simulink model "IEEE_BUS_68_AGC"  (R2025a)
settings: Solver=ode23tb  StartTime=0.0  StopTime=150  FixedStep=Ts  MaxStep=0.0001  RelTol=1e-3
PreLoadFcn:
  | PSSMODEL=1;
  | LPSS=0;
  | WAPSS=0;
  | WAPSS2=0;
  | Ts=50e-5;
InitFcn:
  | PSSMODEL=1;
  | LPSS=0;
  | WAPSS=0;
  | WAPSS2=0;
  | Ts=50e-5;
  | 
  | % Required data to 68 Bus benchmark
  | % clear
  | % clc
  | % Definition for the columns
  | % system base =100 MVA
  | 
  | %% Line data Format (line)
  | % All values are given on the same system base MVA
  | % 1: From bus
  | % 2: To bus
  | % 3: Resistance (pu)
  | % 4: Reactance  (pu)
  | % 5: Charge     (pu)
  | % 6: Transformer Tap Amplitute
  | % 7: base MVA
  | % 8: Nomonal Voltage (KV)
  | 
  | %1   2    3        4       5       6        7      8
  | line=[...
  | 1	54	0	     0.0181	  0	      1.025     100    13.8
  | 2	58	0	     0.025	  0	      1.070     100    13.8
  | 3	62	0	     0.02	  0	      1.070     100    13.8
  | 4	19	0.0007	 0.0142	  0	      1.070     100    13.8
  | 5	20	0.0009	 0.018	  0	      1.009     100    13.8
  | 6	22	0	     0.0143	  0	      1.025     100    13.8
  | 7	23	0.0005	 0.0272	  0	      0         100    13.8
  | 8	25	0.0006	 0.0232	  0	      1.025     100    13.8
  | 9	29	0.0008	 0.0156   0	      1.025     100    13.8
  | 10	31	0	     0.026	  0	      1.04      100    13.8
  | 11	32	0	     0.013	  0	      1.04      100    13.8
  | 12	36	0	     0.0075	  0	      1.04      100    13.8
  | 13	17	0	     0.0033	  0	      1.04      100    13.8
  | 14	41	0	     0.0015	  0	      1         100    13.8
  | 15	42	0	     0.0015	  0	      1         100    13.8
  | 16	18	0	     0.003	  0	      1         100    13.8
  | 17	36	0.0005	 0.0045	  0.32	  0         100    138
  | 17	43	0.0005	 0.0276	  0	      0         100    138
  | 18	42	0.004	 0.06	  2.25    0         100    138
  | 18	49	0.0076	 0.1141	  1.16    0	        100    138
  | 18	50	0.0012	 0.0288	  2.06	  0         100    138
  | 20	19	0.0007	 0.0138	  0       1.06	    100    138
  | 19	68	0.0016	 0.0195	  0.304	  0         100    138
  | 21	22	0.0008	 0.014	  0.2565  0	        100    138
  | 21	68	0.0008	 0.0135	  0.2548  0	        100    138
  | 22	23	0.0006	 0.0096	  0.1846  0	        100    138
  | 23	24	0.0022	 0.035	  0.361	  0         100    138
  | 24	68	0.0003	 0.0059	  0.068	  0         100    138
  | 25	26	0.0032	 0.0323	  0.531	  0         100    138
  | 25	54	0.007	 0.0086	  0.146	  0         100    138
  | 26	27	0.0014	 0.0147	  0.2396  0	        100    138
  | 26	28	0.0043	 0.0474	  0.7802  0	        100    138
  | 26	29	0.0057	 0.0625	  1.029	  0         100    138
  | 27	37	0.0013	 0.0173	  0.3216  0	        100    138
  | 27	53	0.032	 0.32	  0.41	  0         100    138
  | ... (+206 lines)
undefined symbols (not defined in the file or in its folder): D1, Delta
libraries: spsPMUPLLBasedPositiveSequenceLib x90, spsRMSLib x73, spsThreePhaseVIMeasurementLib x69, spsLoadFlowBusLib x69, spsThreePhasePISectionLineLib x64, spsThreePhaseParallelRLCLoadLib x35, spsGenericPowerSystemStabilizerLib x32, spsThreePhaseSeriesRLCLoadLib x21, spsThreePhaseTransformerTwoWindingsLib x21, spsSynchronousMachinepuStandardLib x20, spsExcitationSystemLib x16, spsMultiBandPowerSystemStabilizerLib x16
(part 7 of 8)

== system IEEE_BUS_68_AGC/area-5/G15 ==
  "M15: Turbine & Regulators " : Subsystem
  Vref15 : Constant
  gen15 : spsSynchronousMachinepuStandardLib/Synchronous Machine pu Standard  PresetModel=No  MechanicalLoad=Mechanical power Pm  ShowDetailedParameters=on  RotorType=Round  Units=per unit standard parameters  MeasurementBus=off  NominalParameters="[3000*1e6  13.8e3   60 ]"  Reactances1="[mac_con(15,6:8)  mac_con(15,11:13)  mac_con(15,4)]"  Reactances2=[ 1.305, 0.296, 0.252, 0.474, 0.243, 0.18 ]  dAxisTimeConstants=Open-circuit  qAxisTimeConstants=Open-circuit  TimeConstants1=[]  TimeConstants2="[mac_con(15,9:10)  mac_con(15,14:15)]"  TimeConstants3=[]  TimeConstants4=[]  TimeConstants5=[ 1.01, 0.053, 0.1 ]  TimeConstants6=[]  TimeConstants7=[]  TimeConstants8=[]  StatorResistance=mac_con(15,5)  Mechanical="[ mac_con(15,16)  0  4]"  PolePairs=4  InitialConditions=[0 -87.1003 0.333813 0.333813 0.333813 -0.501867 -120.502 119.498 1.00034]  SetSaturation=off  Saturation=[0.6404,0.7127,0.8441,0.9214,0.9956,1.082,1.19,1.316,1.457;0.7,0.7698,0.8872,0.9466,0.9969,1.046,1.1,1.151,1.201]  LoadFlowParameters=[1 830000000 0 0 0]  TsPowergui=0  TsBlock=-1  IterativeModel=Trapezoidal non iterative  IterativeDiscreteModel=Trapezoidal non iterative  BusType=PV  Pref=1000000000  Qref=0  Qmin=-Inf  Qmax=Inf  PLF=0  QLF=0
  A : PMIOPort  Side=Left
  B : PMIOPort  Port=2  Side=Left
  C : PMIOPort  Port=3  Side=Left
  wires:
  "M15: Turbine & Regulators "/1(Pm15) -> gen15/1
  "M15: Turbine & Regulators "/2(Vf15) -> gen15/2
  [PSSmodel] -> "M15: Turbine & Regulators "/4(PSS15)
  Vref15/1 -> "M15: Turbine & Regulators "/3(Vref15)
  gen15/1 -> "M15: Turbine & Regulators "/1(m15)
  [Pref_G15] -> "M15: Turbine & Regulators "/2(Pref15)
  ? -> ?
  ? -> ?
  connections:
  A/RConn1 -- gen15/RConn1
  B/RConn1 -- gen15/RConn2
  C/RConn1 -- gen15/RConn3

== system IEEE_BUS_68_AGC/area-5/G16 ==
  Bus Selector1 : BusSelector  OutputSignals="Mechanical.Rotor speed deviation  dw (pu)"
  "M16: Turbine & Regulators " : Subsystem
  Vref16 : Constant
  gen16 : spsSynchronousMachinepuStandardLib/Synchronous Machine pu Standard  PresetModel=No  MechanicalLoad=Mechanical power Pm  ShowDetailedParameters=on  RotorType=Round  Units=per unit standard parameters  MeasurementBus=off  NominalParameters="[6000*1e6  13.8e3   60 ]"  Reactances1="[mac_con(13,6:8)  mac_con(13,11:13)  mac_con(13,4)]"  Reactances2=[ 1.305, 0.296, 0.252, 0.474, 0.243, 0.18 ]  dAxisTimeConstants=Open-circuit  qAxisTimeConstants=Open-circuit  TimeConstants1=[]  TimeConstants2="[mac_con(13,9:10)  mac_con(13,14:15)]"  TimeConstants3=[]  TimeConstants4=[]  TimeConstants5=[ 1.01, 0.053, 0.1 ]  TimeConstants6=[]  TimeConstants7=[]  TimeConstants8=[]  StatorResistance=mac_con(13,5)  Mechanical="[ mac_con(13,16)  0  4]"  PolePairs=4  InitialConditions=[0 -83.0458 0.584924 0.584924 0.584924 1.77315 -118.227 121.773 1.00142]  SetSaturation=off  Saturation=[0.6404,0.7127,0.8441,0.9214,0.9956,1.082,1.19,1.316,1.457;0.7,0.7698,0.8872,0.9466,0.9969,1.046,1.1,1.151,1.201]  LoadFlowParameters=[1 830000000 0 0 0]  TsPowergui=0  TsBlock=-1  IterativeModel=Trapezoidal non iterative  IterativeDiscreteModel=Trapezoidal non iterative  BusType=PV  Pref=3500000000  Qref=0  Qmin=-Inf  Qmax=Inf  PLF=0  QLF=0
  A : PMIOPort  Side=Left
  B : PMIOPort  Port=2  Side=Left
  C : PMIOPort  Port=3  Side=Left
  tag scope: G16_Goto=global
  wires:
  Vref16/1 -> "M16: Turbine & Regulators "/3(Vref16)
  [PSSmodel] -> "M16: Turbine & Regulators "/4(PSS16)
  "M16: Turbine & Regulators "/2(Vf16) -> gen16/2
  "M16: Turbine & Regulators "/1(Pm16) -> gen16/1
  gen16/1 -> Bus Selector1/1, "M16: Turbine & Regulators "/1(m16)
  Bus Selector1/1 -> [G16_Goto]  "<Rotor speed deviation  dw (pu)>"
  [Pref_G16] -> "M16: Turbine & Regulators "/2(Pref16)
  connections:
  C/RConn1 -- gen16/RConn3
  B/RConn1 -- gen16/RConn2
  A/RConn1 -- gen16/RConn1

== system IEEE_BUS_68_AGC/area-1/gen4/M4: Turbine & Regulators  ==
  note: M4
  m4 : Inport
  Pref4 : Inport  Port=2
  Vref4 : Inport  Port=3
  PSS4 : Inport  Port=4
  Bus Selector : BusSelector  OutputSignals="Mechanical.Rotor speed  wm  (pu),Mechanical.Rotor angle deviation  d_theta (rad),Mechanical.Electrical power  Pe (pu),Mechanical.Rotor speed deviation  dw (pu),Mechanical.Rotor mechanical angle  theta (deg),dq0 components.Stator voltage  vd (pu),dq0 components.Stator voltage  vq (pu),Output reactive power  Qeo (pu)"
  Delta Pa PSS 4 : spsGenericPowerSystemStabilizerLib/Generic Power System Stabilizer  Tsensor=15e-3  K=2.5*1.25  Twashout=1  Tleadlag1=[60e-3 1]  Tleadlag2=[0 0]  VSlimits=[-0.15 0.15]  Vinit=0  Plot_On=off  MagdB_On=on  FreqRange=logspace(-2,2,500)
      settings: LibrarySourceBlock=|
      | sps_lib/Electrical Machines/Synchronous Machine Control/Generic
      | Power System Stabilizer
  Delta w PSS (Kundur) 4 : spsGenericPowerSystemStabilizerLib/Generic Power System Stabilizer  Tsensor=15e-3  K=30  Twashout=10  Tleadlag1=[50e-3 20e-3]  Tleadlag2=[3 5.4]  VSlimits=[-0.15 0.15]  Vinit=0  Plot_On=off  MagdB_On=on  FreqRange=logspace(-2,2,500)
      settings: LibrarySourceBlock=|
      | sps_lib/Electrical Machines/Synchronous Machine Control/Generic
      | Power System Stabilizer
  EXCITATION4 : spsExcitationSystemLib/Excitation System  tr=AVR_Data(4,1)  reg=[ AVR_Data(4,2:3) ]  exc=[ 1, 0 ]  tgr=[ AVR_Data(4,4:5)]  damp=[ 0, 0 ]  sat=[ 0, 0 ]  lim="[ AVR_Data(4,7:8)  0 ]"  v0=[0.997 1.0061]
      settings: LibrarySourceBlock=sps_lib/Electrical Machines/Synchronous Machine Control/Excitation System
  MB-PSS4 : spsMultiBandPowerSystemStabilizerLib/Multi-Band Power System Stabilizer  OperationMode=Simplified settings  Kg=MB(1)  GL=[MB(2) MB(3)]  GI=[MB(4) MB(5)]  GH=[MB(6) MB(7)]  GLd=[66 66 9.4]  TcLF=[1.667 2 0 0 0 0 2 2.4 0 0 0 0 1 1]  GId=[66 66 47.6]  TcIF=[1 1 0.25 0.3 0 0 1 1 0.3 0.36 0 0 0 0]  GHd=[66 66 233]  TcHF="[0.01 0.012 0 0 0 0  0.012 0.0144 0 0 0 0 1 1]"  LIM=[.075 .15 .15 .15]  Plot_On=off  MagdB_On=off  FreqRange=logspace(-2,2,500)
      settings: LibrarySourceBlock=|
      | sps_lib/Electrical Machines/Synchronous Machine Control/Multi-Band
      | Power System Stabilizer
  Multiport Switch1 : MultiPortSwitch  Inputs=4  SaturateOnIntegerOverflow=off
  PSS model3 : Constant  Value=0
  PSS model4 : Constant
  Real-Imag to Complex1 : RealImagToComplex
  STG4 : spsSteamTurbineandGovernorLib/Steam Turbine and Governor  gentype=Tandem-compound (single mass)  reg1="[ 1  0.05    0 ]"  reg2="[ 0.001  0.15 ]"  reg3="[ -0.1  0.1  0  4.496 ]"  N=Ns  turb1="[ 0  10   3.3   0.5   ]"  turb2="[   0   0.36    0.36   0.28   ]"  HA="[ 0.046  1.430  1.465   0.192 ]"  KA="[ 90.44  53.88  64.59   62.94  ]"  DA="[ 0.0115  0.3575  0.3663   0.0137  ]"  ini1=0.632  ini2=[0.779316,-31.4247]
      settings: LibrarySourceBlock=|
      | sps_lib/Electrical Machines/Synchronous Machine Control/Steam Turbine
      | and Governor
  Sum2 : Sum  InputSameDT=on  SaturateOnIntegerOverflow=on  OutDataTypeStr=Inherit: Same as first input
  Sum3 : Sum  Inputs=-+  InputSameDT=on  SaturateOnIntegerOverflow=on  OutDataTypeStr=Inherit: Same as first input
  Terminator3 : Terminator
  Terminator4 : Terminator
  Terminator5 : Terminator
  wref4 : Constant
  Pm4 : Outport  InitialOutput=0
  Vf4 : Outport  Port=2  InitialOutput=0
  tag scope: EFD4=global, Pa4=global, Pe4=global, Q4=global, Vt4=global, d_theta4=global, pss4=global, theta4=global, w4=global
  wires:
  Bus Selector/7 -> EXCITATION4/3, Real-Imag to Complex1/2  "<Stator voltage  vq (pu)>"
  wref4/1 -> STG4/1
  Pref4/1 -> STG4/2
  m4/1 -> Bus Selector/1
  Vref4/1 -> EXCITATION4/1
  EXCITATION4/1 -> Vf4/1, [EFD4]
  Real-Imag to Complex1/1 -> [Vt4]
  Bus Selector/5 -> [theta4]  "<Rotor mechanical angle  theta (deg)>"
  Bus Selector/6 -> EXCITATION4/2, Real-Imag to Complex1/1  "<Stator voltage  vd (pu)>"
  STG4/3 -> Terminator3/1
  STG4/4 -> Sum3/2, Pm4/1
  STG4/2 -> Terminator4/1
  STG4/1 -> Terminator5/1
  Bus Selector/1 -> [w4], STG4/3  "<Rotor speed  wm  (pu)>"
  Bus Selector/2 -> STG4/4, [d_theta4]  "<Rotor angle deviation  d_theta (rad)>"
  Bus Selector/3 -> Sum3/1, [Pe4]  "<Electrical power  Pe (pu)>"
  Bus Selector/4 -> Delta w PSS (Kundur) 4/1, MB-PSS4/1  "<Rotor speed deviation  dw (pu)>"
  Bus Selector/8 -> [Q4]  "<Output reactive power  Qeo (pu)>"
  Sum3/1 -> [Pa4], Delta Pa PSS 4/1  "Pm-Pe"
  Sum2/1 -> Multiport Switch1/1
  PSS model4/1 -> Sum2/2
  Delta Pa PSS 4/1 -> Multiport Switch1/5
  Delta w PSS (Kundur) 4/1 -> Multiport Switch1/4
  MB-PSS4/1 -> Multiport Switch1/3
  PSS model3/1 -> Multiport Switch1/2
  Multiport Switch1/1 -> [pss4], EXCITATION4/4
  PSS4/1 -> Sum2/1

== system IEEE_BUS_68_AGC/area-1/gen5/M5: Turbine & Regulators  ==
  note: M5
  m5 : Inport
  Pref5 : Inport  Port=2
  Vref5 : Inport  Port=3
  PSS5 : Inport  Port=4
  Bus Selector : BusSelector  OutputSignals="Mechanical.Rotor speed  wm  (pu),Mechanical.Rotor angle deviation  d_theta (rad),Mechanical.Electrical power  Pe (pu),Mechanical.Rotor speed deviation  dw (pu),Mechanical.Rotor mechanical angle  theta (deg),dq0 components.Stator voltage  vd (pu),dq0 components.Stator voltage  vq (pu),Output reactive power  Qeo (pu)"
  Delta Pa PSS 5 : spsGenericPowerSystemStabilizerLib/Generic Power System Stabilizer  Tsensor=15e-3  K=2.5*1.25  Twashout=1  Tleadlag1=[60e-3 1]  Tleadlag2=[0 0]  VSlimits=[-0.15 0.15]  Vinit=0  Plot_On=off  MagdB_On=on  FreqRange=logspace(-2,2,500)
      settings: LibrarySourceBlock=|
      | sps_lib/Electrical Machines/Synchronous Machine Control/Generic
      | Power System Stabilizer
  Delta w PSS (Kundur) 5 : spsGenericPowerSystemStabilizerLib/Generic Power System Stabilizer  Tsensor=15e-3  K=30  Twashout=10  Tleadlag1=[50e-3 20e-3]  Tleadlag2=[3 5.4]  VSlimits=[-0.15 0.15]  Vinit=0  Plot_On=off  MagdB_On=on  FreqRange=logspace(-2,2,500)
      settings: LibrarySourceBlock=|
      | sps_lib/Electrical Machines/Synchronous Machine Control/Generic
      | Power System Stabilizer
  EXCITATION5 : spsExcitationSystemLib/Excitation System  tr=AVR_Data(4,1)  reg=[ AVR_Data(4,2:3) ]  exc=[ 1, 0 ]  tgr=[ AVR_Data(4,4:5)]  damp=[ 0, 0 ]  sat=[ 0, 0 ]  lim="[ AVR_Data(4,7:8)  0 ]"  v0=[1.011 1.0593]
      settings: LibrarySourceBlock=sps_lib/Electrical Machines/Synchronous Machine Control/Excitation System
  MB-PSS5 : spsMultiBandPowerSystemStabilizerLib/Multi-Band Power System Stabilizer  OperationMode=Simplified settings  Kg=MB(1)  GL=[MB(2) MB(3)]  GI=[MB(4) MB(5)]  GH=[MB(6) MB(7)]  GLd=[66 66 9.4]  TcLF=[1.667 2 0 0 0 0 2 2.4 0 0 0 0 1 1]  GId=[66 66 47.6]  TcIF=[1 1 0.25 0.3 0 0 1 1 0.3 0.36 0 0 0 0]  GHd=[66 66 233]  TcHF="[0.01 0.012 0 0 0 0  0.012 0.0144 0 0 0 0 1 1]"  LIM=[.075 .15 .15 .15]  Plot_On=off  MagdB_On=off  FreqRange=logspace(-2,2,500)
      settings: LibrarySourceBlock=|
      | sps_lib/Electrical Machines/Synchronous Machine Control/Multi-Band
      | Power System Stabilizer
  Multiport Switch1 : MultiPortSwitch  Inputs=4  SaturateOnIntegerOverflow=off
  PSS model3 : Constant  Value=0
  PSS model4 : Constant
  Real-Imag to Complex1 : RealImagToComplex
  STG5 : spsSteamTurbineandGovernorLib/Steam Turbine and Governor  gentype=Tandem-compound (single mass)  reg1="[ 1  0.05    0 ]"  reg2="[ 0.001  0.15 ]"  reg3="[ -0.1  0.1  0  4.496 ]"  N=Ns  turb1="[ 0  10   3.3   0.5   ]"  turb2="[   0   0.36    0.36   0.28   ]"  HA="[ 0.046  1.430  1.465   0.192 ]"  KA="[ 90.44  53.88  64.59   62.94  ]"  DA="[ 0.0115  0.3575  0.3663   0.0137  ]"  ini1=0.505  ini2=[0.779316,-31.4247]
      settings: LibrarySourceBlock=|
      | sps_lib/Electrical Machines/Synchronous Machine Control/Steam Turbine
      | and Governor
  Sum2 : Sum  InputSameDT=on  SaturateOnIntegerOverflow=on  OutDataTypeStr=Inherit: Same as first input
  Sum3 : Sum  Inputs=-+  InputSameDT=on  SaturateOnIntegerOverflow=on  OutDataTypeStr=Inherit: Same as first input
  Terminator3 : Terminator
  Terminator4 : Terminator
  Terminator5 : Terminator
  wref5 : Constant
  Pm4 : Outport  InitialOutput=0
  Vf5 : Outport  Port=2  InitialOutput=0
  tag scope: EFD5=global, Pa5=global, Pe5=global, Q5=global, Vt5=global, d_theta5=global, pss5=global, theta5=global, w5=global
  wires:
  PSS5/1 -> Sum2/1
  Multiport Switch1/1 -> EXCITATION5/4, [pss5]
  PSS model3/1 -> Multiport Switch1/2
  MB-PSS5/1 -> Multiport Switch1/3
  Delta w PSS (Kundur) 5/1 -> Multiport Switch1/4
  Delta Pa PSS 5/1 -> Multiport Switch1/5
  PSS model4/1 -> Sum2/2
  Sum2/1 -> Multiport Switch1/1
  Sum3/1 -> Delta Pa PSS 5/1, [Pa5]  "Pm-Pe"
  Bus Selector/8 -> [Q5]  "<Output reactive power  Qeo (pu)>"
  Bus Selector/4 -> MB-PSS5/1, Delta w PSS (Kundur) 5/1  "<Rotor speed deviation  dw (pu)>"
  Bus Selector/3 -> [Pe5], Sum3/1  "<Electrical power  Pe (pu)>"
  Bus Selector/2 -> [d_theta5], STG5/4  "<Rotor angle deviation  d_theta (rad)>"
  Bus Selector/1 -> STG5/3, [w5]  "<Rotor speed  wm  (pu)>"
  STG5/1 -> Terminator5/1
  STG5/2 -> Terminator4/1
  STG5/4 -> Pm4/1, Sum3/2
  STG5/3 -> Terminator3/1
  Bus Selector/6 -> Real-Imag to Complex1/1, EXCITATION5/2  "<Stator voltage  vd (pu)>"
  Bus Selector/5 -> [theta5]  "<Rotor mechanical angle  theta (deg)>"
  Real-Imag to Complex1/1 -> [Vt5]
  EXCITATION5/1 -> [EFD5], Vf5/1
  Vref5/1 -> EXCITATION5/1
  m5/1 -> Bus Selector/1
  Pref5/1 -> STG5/2
  wref5/1 -> STG5/1
  Bus Selector/7 -> Real-Imag to Complex1/2, EXCITATION5/3  "<Stator voltage  vq (pu)>"

== system IEEE_BUS_68_AGC/area-1/gen6/M6: Turbine & Regulators  ==
  note: M6
  m6 : Inport
  Pref6 : Inport  Port=2
  Vref6 : Inport  Port=3
  PSS6 : Inport  Port=4
  Bus Selector : BusSelector  OutputSignals="Mechanical.Rotor speed  wm  (pu),Mechanical.Rotor angle deviation  d_theta (rad),Mechanical.Electrical power  Pe (pu),Mechanical.Rotor speed deviation  dw (pu),Mechanical.Rotor mechanical angle  theta (deg),dq0 components.Stator voltage  vd (pu),dq0 components.Stator voltage  vq (pu),Output reactive power  Qeo (pu)"
  Delta Pa PSS 6 : spsGenericPowerSystemStabilizerLib/Generic Power System Stabilizer  Tsensor=15e-3  K=2.5*1.25  Twashout=1  Tleadlag1=[60e-3 1]  Tleadlag2=[0 0]  VSlimits=[-0.15 0.15]  Vinit=0  Plot_On=off  MagdB_On=on  FreqRange=logspace(-2,2,500)
      settings: LibrarySourceBlock=|
      | sps_lib/Electrical Machines/Synchronous Machine Control/Generic
      | Power System Stabilizer
  Delta w PSS (Kundur) 6 : spsGenericPowerSystemStabilizerLib/Generic Power System Stabilizer  Tsensor=15e-3  K=30  Twashout=10  Tleadlag1=[50e-3 20e-3]  Tleadlag2=[3 5.4]  VSlimits=[-0.15 0.15]  Vinit=0  Plot_On=off  MagdB_On=on  FreqRange=logspace(-2,2,500)
      settings: LibrarySourceBlock=|
      | sps_lib/Electrical Machines/Synchronous Machine Control/Generic
      | Power System Stabilizer
  EXCITATION6 : spsExcitationSystemLib/Excitation System  tr=AVR_Data(4,1)  reg=[ AVR_Data(4,2:3) ]  exc=[ 1, 0 ]  tgr=[ AVR_Data(4,4:5)]  damp=[ 0, 0 ]  sat=[ 0, 0 ]  lim="[ AVR_Data(4,7:8)  0 ]"  v0=[1.05 1.103]
      settings: LibrarySourceBlock=sps_lib/Electrical Machines/Synchronous Machine Control/Excitation System
  MB-PSS6 : spsMultiBandPowerSystemStabilizerLib/Multi-Band Power System Stabilizer  OperationMode=Simplified settings  Kg=MB(1)  GL=[MB(2) MB(3)]  GI=[MB(4) MB(5)]  GH=[MB(6) MB(7)]  GLd=[66 66 9.4]  TcLF=[1.667 2 0 0 0 0 2 2.4 0 0 0 0 1 1]  GId=[66 66 47.6]  TcIF=[1 1 0.25 0.3 0 0 1 1 0.3 0.36 0 0 0 0]  GHd=[66 66 233]  TcHF="[0.01 0.012 0 0 0 0  0.012 0.0144 0 0 0 0 1 1]"  LIM=[.075 .15 .15 .15]  Plot_On=off  MagdB_On=off  FreqRange=logspace(-2,2,500)
      settings: LibrarySourceBlock=|
      | sps_lib/Electrical Machines/Synchronous Machine Control/Multi-Band
      | Power System Stabilizer
  Multiport Switch1 : MultiPortSwitch  Inputs=4  SaturateOnIntegerOverflow=off
  PSS model3 : Constant  Value=0
  PSS model4 : Constant
  Real-Imag to Complex1 : RealImagToComplex
  STG6 : spsSteamTurbineandGovernorLib/Steam Turbine and Governor  gentype=Tandem-compound (single mass)  reg1="[ 1  0.05    0 ]"  reg2="[ 0.001  0.15 ]"  reg3="[ -0.1  0.1  0  4.496 ]"  N=Ns  turb1="[ 0  10   3.3   0.5   ]"  turb2="[   0   0.36    0.36   0.28   ]"  HA="[ 0.046  1.430  1.465   0.192 ]"  KA="[ 90.44  53.88  64.59   62.94  ]"  DA="[ 0.0115  0.3575  0.3663   0.0137  ]"  ini1=0.7  ini2=[0.779316,-31.4247]
      settings: LibrarySourceBlock=|
      | sps_lib/Electrical Machines/Synchronous Machine Control/Steam Turbine
      | and Governor
  Sum2 : Sum  InputSameDT=on  SaturateOnIntegerOverflow=on  OutDataTypeStr=Inherit: Same as first input
  Sum3 : Sum  Inputs=-+  InputSameDT=on  SaturateOnIntegerOverflow=on  OutDataTypeStr=Inherit: Same as first input
  Terminator3 : Terminator
  Terminator4 : Terminator
  Terminator5 : Terminator
  wref6 : Constant
  Pm6 : Outport  InitialOutput=0
  Vf6 : Outport  Port=2  InitialOutput=0
  tag scope: EFD6=global, Pa6=global, Pe6=global, Q6=global, Vt6=global, d_theta6=global, pss6=global, theta6=global, w6=global
  wires:
  PSS6/1 -> Sum2/1
  Multiport Switch1/1 -> EXCITATION6/4, [pss6]
  PSS model3/1 -> Multiport Switch1/2
  MB-PSS6/1 -> Multiport Switch1/3
  Delta w PSS (Kundur) 6/1 -> Multiport Switch1/4
  Delta Pa PSS 6/1 -> Multiport Switch1/5
  PSS model4/1 -> Sum2/2
  Sum2/1 -> Multiport Switch1/1
  Sum3/1 -> Delta Pa PSS 6/1, [Pa6]  "Pm-Pe"
  Bus Selector/8 -> [Q6]  "<Output reactive power  Qeo (pu)>"
  Bus Selector/4 -> MB-PSS6/1, Delta w PSS (Kundur) 6/1  "<Rotor speed deviation  dw (pu)>"
  Bus Selector/3 -> [Pe6], Sum3/1  "<Electrical power  Pe (pu)>"
  Bus Selector/2 -> [d_theta6], STG6/4  "<Rotor angle deviation  d_theta (rad)>"
  Bus Selector/1 -> STG6/3, [w6]  "<Rotor speed  wm  (pu)>"
  STG6/1 -> Terminator5/1
  STG6/2 -> Terminator4/1
  STG6/4 -> Pm6/1, Sum3/2
  STG6/3 -> Terminator3/1
  Bus Selector/6 -> Real-Imag to Complex1/1, EXCITATION6/2  "<Stator voltage  vd (pu)>"
  Bus Selector/5 -> [theta6]  "<Rotor mechanical angle  theta (deg)>"
  Real-Imag to Complex1/1 -> [Vt6]
  EXCITATION6/1 -> [EFD6], Vf6/1
  Vref6/1 -> EXCITATION6/1
  m6/1 -> Bus Selector/1
  Pref6/1 -> STG6/2
  wref6/1 -> STG6/1
  Bus Selector/7 -> Real-Imag to Complex1/2, EXCITATION6/3  "<Stator voltage  vq (pu)>"

== system IEEE_BUS_68_AGC/area-1/gen7/M7: Turbine & Regulators  ==
  note: M7
  m7 : Inport
  Pref7 : Inport  Port=2
  Vref7 : Inport  Port=3
  PSS7 : Inport  Port=4
  Bus Selector : BusSelector  OutputSignals="Mechanical.Rotor speed  wm  (pu),Mechanical.Rotor angle deviation  d_theta (rad),Mechanical.Electrical power  Pe (pu),Mechanical.Rotor speed deviation  dw (pu),Mechanical.Rotor mechanical angle  theta (deg),dq0 components.Stator voltage  vd (pu),dq0 components.Stator voltage  vq (pu),Output reactive power  Qeo (pu)"
  Delta Pa PSS 7 : spsGenericPowerSystemStabilizerLib/Generic Power System Stabilizer  Tsensor=15e-3  K=2.5*1.25  Twashout=1  Tleadlag1=[60e-3 1]  Tleadlag2=[0 0]  VSlimits=[-0.15 0.15]  Vinit=0  Plot_On=off  MagdB_On=on  FreqRange=logspace(-2,2,500)
      settings: LibrarySourceBlock=|
      | sps_lib/Electrical Machines/Synchronous Machine Control/Generic
      | Power System Stabilizer
  Delta w PSS (Kundur) 7 : spsGenericPowerSystemStabilizerLib/Generic Power System Stabilizer  Tsensor=15e-3  K=30  Twashout=10  Tleadlag1=[50e-3 20e-3]  Tleadlag2=[3 5.4]  VSlimits=[-0.15 0.15]  Vinit=0  Plot_On=off  MagdB_On=on  FreqRange=logspace(-2,2,500)
      settings: LibrarySourceBlock=|
      | sps_lib/Electrical Machines/Synchronous Machine Control/Generic
      | Power System Stabilizer
  EXCITATION7 : spsExcitationSystemLib/Excitation System  tr=AVR_Data(4,1)  reg=[ AVR_Data(4,2:3) ]  exc=[ 1, 0 ]  tgr=[ AVR_Data(4,4:5)]  damp=[ 0, 0 ]  sat=[ 0, 0 ]  lim="[ AVR_Data(4,7:8)  0 ]"  v0=[1.063 1.1185]
      settings: LibrarySourceBlock=sps_lib/Electrical Machines/Synchronous Machine Control/Excitation System
  MB-PSS7 : spsMultiBandPowerSystemStabilizerLib/Multi-Band Power System Stabilizer  OperationMode=Simplified settings  Kg=MB(1)  GL=[MB(2) MB(3)]  GI=[MB(4) MB(5)]  GH=[MB(6) MB(7)]  GLd=[66 66 9.4]  TcLF=[1.667 2 0 0 0 0 2 2.4 0 0 0 0 1 1]  GId=[66 66 47.6]  TcIF=[1 1 0.25 0.3 0 0 1 1 0.3 0.36 0 0 0 0]  GHd=[66 66 233]  TcHF="[0.01 0.012 0 0 0 0  0.012 0.0144 0 0 0 0 1 1]"  LIM=[.075 .15 .15 .15]  Plot_On=off  MagdB_On=off  FreqRange=logspace(-2,2,500)
      settings: LibrarySourceBlock=|
      | sps_lib/Electrical Machines/Synchronous Machine Control/Multi-Band
      | Power System Stabilizer
  Multiport Switch1 : MultiPortSwitch  Inputs=4  SaturateOnIntegerOverflow=off
  PSS model3 : Constant  Value=0
  PSS model4 : Constant
  Real-Imag to Complex1 : RealImagToComplex
  STG7 : spsSteamTurbineandGovernorLib/Steam Turbine and Governor  gentype=Tandem-compound (single mass)  reg1="[ 1  0.05    0 ]"  reg2="[ 0.001  0.15 ]"  reg3="[ -0.1  0.1  0  4.496 ]"  N=Ns  turb1="[ 0  10   3.3   0.5   ]"  turb2="[   0   0.36    0.36   0.28   ]"  HA="[ 0.046  1.430  1.465   0.192 ]"  KA="[ 90.44  53.88  64.59   62.94  ]"  DA="[ 0.0115  0.3575  0.3663   0.0137  ]"  ini1=0.56  ini2=[0.779316,-31.4247]
      settings: LibrarySourceBlock=|
      | sps_lib/Electrical Machines/Synchronous Machine Control/Steam Turbine
      | and Governor
  Sum2 : Sum  InputSameDT=on  SaturateOnIntegerOverflow=on  OutDataTypeStr=Inherit: Same as first input
  Sum3 : Sum  Inputs=-+  InputSameDT=on  SaturateOnIntegerOverflow=on  OutDataTypeStr=Inherit: Same as first input
  Terminator3 : Terminator
  Terminator4 : Terminator
  Terminator5 : Terminator
  wref7 : Constant
  Pm7 : Outport  InitialOutput=0
  Vf7 : Outport  Port=2  InitialOutput=0
  tag scope: EFD7=global, Pa7=global, Pe7=global, Q7=global, Vt7=global, d_theta7=global, pss7=global, theta7=global, w7=global
  wires:
  PSS7/1 -> Sum2/1
  Multiport Switch1/1 -> EXCITATION7/4, [pss7]
  PSS model3/1 -> Multiport Switch1/2
  MB-PSS7/1 -> Multiport Switch1/3
  Delta w PSS (Kundur) 7/1 -> Multiport Switch1/4
  Delta Pa PSS 7/1 -> Multiport Switch1/5
  PSS model4/1 -> Sum2/2
  Sum2/1 -> Multiport Switch1/1
  Sum3/1 -> Delta Pa PSS 7/1, [Pa7]  "Pm-Pe"
  Bus Selector/8 -> [Q7]  "<Output reactive power  Qeo (pu)>"
  Bus Selector/4 -> MB-PSS7/1, Delta w PSS (Kundur) 7/1  "<Rotor speed deviation  dw (pu)>"
  Bus Selector/3 -> [Pe7], Sum3/1  "<Electrical power  Pe (pu)>"
  Bus Selector/2 -> [d_theta7], STG7/4  "<Rotor angle deviation  d_theta (rad)>"
  Bus Selector/1 -> STG7/3, [w7]  "<Rotor speed  wm  (pu)>"
  STG7/1 -> Terminator5/1
  STG7/2 -> Terminator4/1
  STG7/4 -> Pm7/1, Sum3/2
  STG7/3 -> Terminator3/1
  Bus Selector/6 -> Real-Imag to Complex1/1, EXCITATION7/2  "<Stator voltage  vd (pu)>"
  Bus Selector/5 -> [theta7]  "<Rotor mechanical angle  theta (deg)>"
  Real-Imag to Complex1/1 -> [Vt7]
  EXCITATION7/1 -> [EFD7], Vf7/1
  Vref7/1 -> EXCITATION7/1
  m7/1 -> Bus Selector/1
  Pref7/1 -> STG7/2
  wref7/1 -> STG7/1
  Bus Selector/7 -> Real-Imag to Complex1/2, EXCITATION7/3  "<Stator voltage  vq (pu)>"

== system IEEE_BUS_68_AGC/area-2/G2/M2: Turbine & Regulators  ==
  note: M2
  m2 : Inport
  Pref2 : Inport  Port=2
  Vref2 : Inport  Port=3
  PSS2 : Inport  Port=4
  Bus Selector : BusSelector  OutputSignals="Mechanical.Rotor speed  wm  (pu),Mechanical.Rotor angle deviation  d_theta (rad),Mechanical.Electrical power  Pe (pu),Mechanical.Rotor speed deviation  dw (pu),Mechanical.Rotor mechanical angle  theta (deg),dq0 components.Stator voltage  vd (pu),dq0 components.Stator voltage  vq (pu),Output reactive power  Qeo (pu)"
  "Delta Pa PSS 2 " : spsGenericPowerSystemStabilizerLib/Generic Power System Stabilizer  Tsensor=15e-3  K=2.5*1.25  Twashout=1  Tleadlag1=[60e-3 1]  Tleadlag2=[0 0]  VSlimits=[-0.15 0.15]  Vinit=0  Plot_On=off  MagdB_On=on  FreqRange=logspace(-2,2,500)
      settings: LibrarySourceBlock=|
      | sps_lib/Electrical Machines/Synchronous Machine Control/Generic
      | Power System Stabilizer
  Delta w PSS (Kundur) 2 : spsGenericPowerSystemStabilizerLib/Generic Power System Stabilizer  Tsensor=15e-3  K=30  Twashout=10  Tleadlag1=[50e-3 20e-3]  Tleadlag2=[3 5.4]  VSlimits=[-0.15 0.15]  Vinit=0  Plot_On=off  MagdB_On=on  FreqRange=logspace(-2,2,500)
      settings: LibrarySourceBlock=|
      | sps_lib/Electrical Machines/Synchronous Machine Control/Generic
      | Power System Stabilizer
  EXCITATION2 : spsExcitationSystemLib/Excitation System  tr=AVR_Data(2,1)  reg=[ AVR_Data(2,2:3) ]  exc=[ 1, 0 ]  tgr=[ AVR_Data(2,4:5)]  damp=[ 0, 0 ]  sat=[ 0, 0 ]  lim="[ AVR_Data(2,7:8)  0 ]"  v0=[0.98 1.019]
      settings: LibrarySourceBlock=sps_lib/Electrical Machines/Synchronous Machine Control/Excitation System
  MB-PSS2 : spsMultiBandPowerSystemStabilizerLib/Multi-Band Power System Stabilizer  OperationMode=Simplified settings  Kg=MB(1)  GL=[MB(2) MB(3)]  GI=[MB(4) MB(5)]  GH=[MB(6) MB(7)]  GLd=[66 66 9.4]  TcLF=[1.667 2 0 0 0 0 2 2.4 0 0 0 0 1 1]  GId=[66 66 47.6]  TcIF=[1 1 0.25 0.3 0 0 1 1 0.3 0.36 0 0 0 0]  GHd=[66 66 233]  TcHF="[0.01 0.012 0 0 0 0  0.012 0.0144 0 0 0 0 1 1]"  LIM=[.075 .15 .15 .15]  Plot_On=off  MagdB_On=off  FreqRange=logspace(-2,2,500)
      settings: LibrarySourceBlock=|
      | sps_lib/Electrical Machines/Synchronous Machine Control/Multi-Band
      | Power System Stabilizer
  Multiport Switch1 : MultiPortSwitch  Inputs=4  SaturateOnIntegerOverflow=off
  PSS model3 : Constant  Value=0
  PSS model4 : Constant
  Real-Imag to Complex1 : RealImagToComplex
  STG2 : spsSteamTurbineandGovernorLib/Steam Turbine and Governor  gentype=Tandem-compound (single mass)  reg1="[ 1  0.05    0 ]"  reg2="[ 0.001  0.15 ]"  reg3="[ -0.1  0.1  0  4.496 ]"  N=Ns  turb1="[ 0  10   3.3   0.5   ]"  turb2="[   0   0.36    0.36   0.28   ]"  HA="[ 0.046  1.430  1.465   0.192 ]"  KA="[ 90.44  53.88  64.59   62.94  ]"  DA="[ 0.0115  0.3575  0.3663   0.0137  ]"  ini1=0.545  ini2=[0.779316,-31.4247]
      settings: LibrarySourceBlock=|
      | sps_lib/Electrical Machines/Synchronous Machine Control/Steam Turbine
      | and Governor
  Sum2 : Sum  InputSameDT=on  SaturateOnIntegerOverflow=on  OutDataTypeStr=Inherit: Same as first input
  Sum3 : Sum  Inputs=-+  InputSameDT=on  SaturateOnIntegerOverflow=on  OutDataTypeStr=Inherit: Same as first input
  Terminator3 : Terminator
  Terminator4 : Terminator
  Terminator5 : Terminator
  wref2 : Constant
  Pm2 : Outport  InitialOutput=0
  Vf2 : Outport  Port=2  InitialOutput=0
  tag scope: EFD2=global, Pa2=global, Pe2=global, Q2=global, Vt2=global, d_theta2=global, pss2=global, theta2=global, w2=global
  wires:
  Bus Selector/7 -> EXCITATION2/3, Real-Imag to Complex1/2  "<Stator voltage  vq (pu)>"
  wref2/1 -> STG2/1
  Pref2/1 -> STG2/2
  m2/1 -> Bus Selector/1
  Vref2/1 -> EXCITATION2/1
  EXCITATION2/1 -> Vf2/1, [EFD2]
  Real-Imag to Complex1/1 -> [Vt2]
  Bus Selector/5 -> [theta2]  "<Rotor mechanical angle  theta (deg)>"
  Bus Selector/6 -> EXCITATION2/2, Real-Imag to Complex1/1  "<Stator voltage  vd (pu)>"
  STG2/3 -> Terminator3/1
  STG2/4 -> Sum3/2, Pm2/1
  STG2/2 -> Terminator4/1
  STG2/1 -> Terminator5/1
  Bus Selector/1 -> [w2], STG2/3  "<Rotor speed  wm  (pu)>"
  Bus Selector/2 -> STG2/4, [d_theta2]  "<Rotor angle deviation  d_theta (rad)>"
  Bus Selector/3 -> Sum3/1, [Pe2]  "<Electrical power  Pe (pu)>"
  Bus Selector/4 -> Delta w PSS (Kundur) 2/1, MB-PSS2/1  "<Rotor speed deviation  dw (pu)>"
  Bus Selector/8 -> [Q2]  "<Output reactive power  Qeo (pu)>"
  Sum3/1 -> [Pa2], "Delta Pa PSS 2 "/1  "Pm-Pe"
  Sum2/1 -> Multiport Switch1/1
  PSS model4/1 -> Sum2/2
  "Delta Pa PSS 2 "/1 -> Multiport Switch1/5
  Delta w PSS (Kundur) 2/1 -> Multiport Switch1/4
  MB-PSS2/1 -> Multiport Switch1/3
  PSS model3/1 -> Multiport Switch1/2
  Multiport Switch1/1 -> [pss2], EXCITATION2/4
  PSS2/1 -> Sum2/1

== system IEEE_BUS_68_AGC/area-2/G3/M3: Turbine & Regulators  ==
  note: M3
  m3 : Inport
  Pref3 : Inport  Port=2
  Vref3 : Inport  Port=3
  PSS3 : Inport  Port=4
  Bus Selector : BusSelector  OutputSignals="Mechanical.Rotor speed  wm  (pu),Mechanical.Rotor angle deviation  d_theta (rad),Mechanical.Electrical power  Pe (pu),Mechanical.Rotor speed deviation  dw (pu),Mechanical.Rotor mechanical angle  theta (deg),dq0 components.Stator voltage  vd (pu),dq0 components.Stator voltage  vq (pu),Output reactive power  Qeo (pu)"
  "Delta Pa PSS 3 " : spsGenericPowerSystemStabilizerLib/Generic Power System Stabilizer  Tsensor=15e-3  K=2.5*1.25  Twashout=1  Tleadlag1=[60e-3 1]  Tleadlag2=[0 0]  VSlimits=[-0.15 0.15]  Vinit=0  Plot_On=off  MagdB_On=on  FreqRange=logspace(-2,2,500)
      settings: LibrarySourceBlock=|
      | sps_lib/Electrical Machines/Synchronous Machine Control/Generic
      | Power System Stabilizer
  Delta w PSS (Kundur) 3 : spsGenericPowerSystemStabilizerLib/Generic Power System Stabilizer  Tsensor=15e-3  K=30  Twashout=10  Tleadlag1=[50e-3 20e-3]  Tleadlag2=[3 5.4]  VSlimits=[-0.15 0.15]  Vinit=0  Plot_On=off  MagdB_On=on  FreqRange=logspace(-2,2,500)
      settings: LibrarySourceBlock=|
      | sps_lib/Electrical Machines/Synchronous Machine Control/Generic
      | Power System Stabilizer
  EXCITATION3 : spsExcitationSystemLib/Excitation System  tr=AVR_Data(3,1)  reg=[ AVR_Data(3,2:3) ]  exc=[ 1, 0 ]  tgr=[ AVR_Data(3,4:5)]  damp=[ 0, 0 ]  sat=[ 0, 0 ]  lim="[ AVR_Data(3,7:8)  0 ]"  v0=[0.983 0.98897]
      settings: LibrarySourceBlock=sps_lib/Electrical Machines/Synchronous Machine Control/Excitation System
  MB-PSS3 : spsMultiBandPowerSystemStabilizerLib/Multi-Band Power System Stabilizer  OperationMode=Simplified settings  Kg=MB(1)  GL=[MB(2) MB(3)]  GI=[MB(4) MB(5)]  GH=[MB(6) MB(7)]  GLd=[66 66 9.4]  TcLF=[1.667 2 0 0 0 0 2 2.4 0 0 0 0 1 1]  GId=[66 66 47.6]  TcIF=[1 1 0.25 0.3 0 0 1 1 0.3 0.36 0 0 0 0]  GHd=[66 66 233]  TcHF="[0.01 0.012 0 0 0 0  0.012 0.0144 0 0 0 0 1 1]"  LIM=[.075 .15 .15 .15]  Plot_On=off  MagdB_On=off  FreqRange=logspace(-2,2,500)
      settings: LibrarySourceBlock=|
      | sps_lib/Electrical Machines/Synchronous Machine Control/Multi-Band
      | Power System Stabilizer
  Multiport Switch1 : MultiPortSwitch  Inputs=4  SaturateOnIntegerOverflow=off
  PSS model3 : Constant  Value=0
  PSS model4 : Constant
  Real-Imag to Complex1 : RealImagToComplex
  STG3 : spsSteamTurbineandGovernorLib/Steam Turbine and Governor  gentype=Tandem-compound (single mass)  reg1="[ 1  0.05    0 ]"  reg2="[ 0.001  0.15 ]"  reg3="[ -0.1  0.1  0  4.496 ]"  N=Ns  turb1="[ 0  10   3.3   0.5   ]"  turb2="[   0   0.36    0.36   0.28   ]"  HA="[ 0.046  1.430  1.465   0.192 ]"  KA="[ 90.44  53.88  64.59   62.94  ]"  DA="[ 0.0115  0.3575  0.3663   0.0137  ]"  ini1=0.325  ini2=[0.779316,-31.4247]
      settings: LibrarySourceBlock=|
      | sps_lib/Electrical Machines/Synchronous Machine Control/Steam Turbine
      | and Governor
  Sum2 : Sum  InputSameDT=on  SaturateOnIntegerOverflow=on  OutDataTypeStr=Inherit: Same as first input
  Sum3 : Sum  Inputs=-+  InputSameDT=on  SaturateOnIntegerOverflow=on  OutDataTypeStr=Inherit: Same as first input
  Terminator3 : Terminator
  Terminator4 : Terminator
  Terminator5 : Terminator
  wref3 : Constant
  Pm3 : Outport  InitialOutput=0
  Vf3 : Outport  Port=2  InitialOutput=0
  tag scope: EFD3=global, Pa3=global, Pe3=global, Q3=global, Vt3=global, d_theta3=global, pss3=global, theta3=global, w3=global
  wires:
  PSS3/1 -> Sum2/1
  Multiport Switch1/1 -> EXCITATION3/4, [pss3]
  PSS model3/1 -> Multiport Switch1/2
  MB-PSS3/1 -> Multiport Switch1/3
  Delta w PSS (Kundur) 3/1 -> Multiport Switch1/4
  "Delta Pa PSS 3 "/1 -> Multiport Switch1/5
  PSS model4/1 -> Sum2/2
  Sum2/1 -> Multiport Switch1/1
  Sum3/1 -> "Delta Pa PSS 3 "/1, [Pa3]  "Pm-Pe"
  Bus Selector/8 -> [Q3]  "<Output reactive power  Qeo (pu)>"
  Bus Selector/4 -> MB-PSS3/1, Delta w PSS (Kundur) 3/1  "<Rotor speed deviation  dw (pu)>"
  Bus Selector/3 -> [Pe3], Sum3/1  "<Electrical power  Pe (pu)>"
  Bus Selector/2 -> [d_theta3], STG3/4  "<Rotor angle deviation  d_theta (rad)>"
  Bus Selector/1 -> STG3/3, [w3]  "<Rotor speed  wm  (pu)>"
  STG3/1 -> Terminator5/1
  STG3/2 -> Terminator4/1
  STG3/4 -> Pm3/1, Sum3/2
  STG3/3 -> Terminator3/1
  Bus Selector/6 -> Real-Imag to Complex1/1, EXCITATION3/2  "<Stator voltage  vd (pu)>"
  Bus Selector/5 -> [theta3]  "<Rotor mechanical angle  theta (deg)>"
  Real-Imag to Complex1/1 -> [Vt3]
  EXCITATION3/1 -> [EFD3], Vf3/1
  Vref3/1 -> EXCITATION3/1
  m3/1 -> Bus Selector/1
  Pref3/1 -> STG3/2
  wref3/1 -> STG3/1
  Bus Selector/7 -> Real-Imag to Complex1/2, EXCITATION3/3  "<Stator voltage  vq (pu)>"

== system IEEE_BUS_68_AGC/area-3/G1/M1: Turbine & Regulators  ==
  note: M1
  m1 : Inport
  Pref1 : Inport  Port=2
  Vref1 : Inport  Port=3
  PSS1 : Inport  Port=4
  Bus Selector : BusSelector  OutputSignals="Mechanical.Rotor speed  wm  (pu),Mechanical.Rotor angle deviation  d_theta (rad),Mechanical.Electrical power  Pe (pu),Mechanical.Rotor speed deviation  dw (pu),Mechanical.Rotor mechanical angle  theta (deg),dq0 components.Stator voltage  vd (pu),dq0 components.Stator voltage  vq (pu),Output reactive power  Qeo (pu)"
  "Delta Pa PSS 1 " : spsGenericPowerSystemStabilizerLib/Generic Power System Stabilizer  Tsensor=15e-3  K=2.5*1.25  Twashout=1  Tleadlag1=[60e-3 1]  Tleadlag2=[0 0]  VSlimits=[-0.15 0.15]  Vinit=0  Plot_On=off  MagdB_On=on  FreqRange=logspace(-2,2,500)
      settings: LibrarySourceBlock=|
      | sps_lib/Electrical Machines/Synchronous Machine Control/Generic
      | Power System Stabilizer
  Delta w PSS (Kundur) 1 : spsGenericPowerSystemStabilizerLib/Generic Power System Stabilizer  Tsensor=15e-3  K=30  Twashout=10  Tleadlag1=[50e-3 20e-3]  Tleadlag2=[3 5.4]  VSlimits=[-0.15 0.15]  Vinit=0  Plot_On=off  MagdB_On=on  FreqRange=logspace(-2,2,500)
      settings: LibrarySourceBlock=|
      | sps_lib/Electrical Machines/Synchronous Machine Control/Generic
      | Power System Stabilizer
  EXCITATION1 : spsExcitationSystemLib/Excitation System  tr=AVR_Data(1,1)  reg=[ AVR_Data(1,2:3) ]  exc=[ 1, 0 ]  tgr=[ AVR_Data(1,4:5)]  damp=[ 0, 0 ]  sat=[ 0, 0 ]  lim="[ AVR_Data(1,7:8)  0 ]"  v0=[1.045 1.0597]
      settings: LibrarySourceBlock=sps_lib/Electrical Machines/Synchronous Machine Control/Excitation System
  MB-PSS1 : spsMultiBandPowerSystemStabilizerLib/Multi-Band Power System Stabilizer  OperationMode=Simplified settings  Kg=MB(1)  GL=[MB(2) MB(3)]  GI=[MB(4) MB(5)]  GH=[MB(6) MB(7)]  GLd=[66 66 9.4]  TcLF=[1.667 2 0 0 0 0 2 2.4 0 0 0 0 1 1]  GId=[66 66 47.6]  TcIF=[1 1 0.25 0.3 0 0 1 1 0.3 0.36 0 0 0 0]  GHd=[66 66 233]  TcHF="[0.01 0.012 0 0 0 0  0.012 0.0144 0 0 0 0 1 1]"  LIM=[.075 .15 .15 .15]  Plot_On=off  MagdB_On=off  FreqRange=logspace(-2,2,500)
      settings: LibrarySourceBlock=|
      | sps_lib/Electrical Machines/Synchronous Machine Control/Multi-Band
      | Power System Stabilizer
  Multiport Switch1 : MultiPortSwitch  Inputs=4  SaturateOnIntegerOverflow=off
  PSS model3 : Constant  Value=0
  PSS model4 : Constant
  Real-Imag to Complex1 : RealImagToComplex
  STG1 : spsSteamTurbineandGovernorLib/Steam Turbine and Governor  gentype=Tandem-compound (single mass)  reg1="[ 1  0.05    0 ]"  reg2="[ 0.001  0.15 ]"  reg3="[ -0.1  0.1  0  4.496 ]"  N=Ns  turb1="[ 0  10   3.3   0.5   ]"  turb2="[   0   0.36    0.36   0.28   ]"  HA="[ 0.046  1.430  1.465   0.192 ]"  KA="[ 90.44  53.88  64.59   62.94  ]"  DA="[ 0.0115  0.3575  0.3663   0.0137  ]"  ini1=0.25  ini2=[0.779316,-31.4247]
      settings: LibrarySourceBlock=|
      | sps_lib/Electrical Machines/Synchronous Machine Control/Steam Turbine
      | and Governor
  Sum2 : Sum  InputSameDT=on  SaturateOnIntegerOverflow=on  OutDataTypeStr=Inherit: Same as first input
  Sum3 : Sum  Inputs=-+  InputSameDT=on  SaturateOnIntegerOverflow=on  OutDataTypeStr=Inherit: Same as first input
  Terminator3 : Terminator
  Terminator4 : Terminator
  Terminator5 : Terminator
  wref1 : Constant
  Pm1 : Outport  InitialOutput=0
  Vf1 : Outport  Port=2  InitialOutput=0
  tag scope: EFD1=global, Pa1=global, Pe1=global, Q1=global, Vt1=global, d_theta1=global, pss1=global, theta1=global, w1=global
  wires:
  PSS1/1 -> Sum2/1
  Multiport Switch1/1 -> EXCITATION1/4, [pss1]
  PSS model3/1 -> Multiport Switch1/2
  MB-PSS1/1 -> Multiport Switch1/3
  Delta w PSS (Kundur) 1/1 -> Multiport Switch1/4
  "Delta Pa PSS 1 "/1 -> Multiport Switch1/5
  PSS model4/1 -> Sum2/2
  Sum2/1 -> Multiport Switch1/1
  Sum3/1 -> "Delta Pa PSS 1 "/1, [Pa1]  "Pm-Pe"
  Bus Selector/8 -> [Q1]  "<Output reactive power  Qeo (pu)>"
  Bus Selector/4 -> MB-PSS1/1, Delta w PSS (Kundur) 1/1  "<Rotor speed deviation  dw (pu)>"
  Bus Selector/3 -> [Pe1], Sum3/1  "<Electrical power  Pe (pu)>"
  Bus Selector/2 -> [d_theta1], STG1/4  "<Rotor angle deviation  d_theta (rad)>"
  Bus Selector/1 -> STG1/3, [w1]  "<Rotor speed  wm  (pu)>"
  STG1/1 -> Terminator5/1
  STG1/2 -> Terminator4/1
  STG1/4 -> Pm1/1, Sum3/2
  STG1/3 -> Terminator3/1
  Bus Selector/6 -> Real-Imag to Complex1/1, EXCITATION1/2  "<Stator voltage  vd (pu)>"
  Bus Selector/5 -> [theta1]  "<Rotor mechanical angle  theta (deg)>"
  Real-Imag to Complex1/1 -> [Vt1]
  EXCITATION1/1 -> [EFD1], Vf1/1
  Vref1/1 -> EXCITATION1/1
  m1/1 -> Bus Selector/1
  Pref1/1 -> STG1/2
  wref1/1 -> STG1/1
  Bus Selector/7 -> Real-Imag to Complex1/2, EXCITATION1/3  "<Stator voltage  vq (pu)>"

== system IEEE_BUS_68_AGC/area-3/G8/M8: Turbine & Regulators  ==
  note: M8
  m8 : Inport
  Pref8 : Inport  Port=2
  Vref8 : Inport  Port=3
  PSS8 : Inport  Port=4
  Bus Selector : BusSelector  OutputSignals="Mechanical.Rotor speed  wm  (pu),Mechanical.Rotor angle deviation  d_theta (rad),Mechanical.Electrical power  Pe (pu),Mechanical.Rotor speed deviation  dw (pu),Mechanical.Rotor mechanical angle  theta (deg),dq0 components.Stator voltage  vd (pu),dq0 components.Stator voltage  vq (pu),Output reactive power  Qeo (pu)"
  "Delta Pa PSS 8 " : spsGenericPowerSystemStabilizerLib/Generic Power System Stabilizer  Tsensor=15e-3  K=2.5*1.25  Twashout=1  Tleadlag1=[60e-3 1]  Tleadlag2=[0 0]  VSlimits=[-0.15 0.15]  Vinit=0  Plot_On=off  MagdB_On=on  FreqRange=logspace(-2,2,500)
      settings: LibrarySourceBlock=|
      | sps_lib/Electrical Machines/Synchronous Machine Control/Generic
      | Power System Stabilizer
  Delta w PSS (Kundur) 8 : spsGenericPowerSystemStabilizerLib/Generic Power System Stabilizer  Tsensor=15e-3  K=30  Twashout=10  Tleadlag1=[50e-3 20e-3]  Tleadlag2=[3 5.4]  VSlimits=[-0.15 0.15]  Vinit=0  Plot_On=off  MagdB_On=on  FreqRange=logspace(-2,2,500)
      settings: LibrarySourceBlock=|
      | sps_lib/Electrical Machines/Synchronous Machine Control/Generic
      | Power System Stabilizer
  EXCITATION8 : spsExcitationSystemLib/Excitation System  tr=AVR_Data(8,1)  reg=[ AVR_Data(8,2:3) ]  exc=[ 1, 0 ]  tgr=[ AVR_Data(8,4:5)]  damp=[ 0, 0 ]  sat=[ 0, 0 ]  lim="[ AVR_Data(8,7:8)  0 ]"  v0=[1.03 1.0417]
      settings: LibrarySourceBlock=sps_lib/Electrical Machines/Synchronous Machine Control/Excitation System
  MB-PSS8 : spsMultiBandPowerSystemStabilizerLib/Multi-Band Power System Stabilizer  OperationMode=Simplified settings  Kg=MB(1)  GL=[MB(2) MB(3)]  GI=[MB(4) MB(5)]  GH=[MB(6) MB(7)]  GLd=[66 66 9.4]  TcLF=[1.667 2 0 0 0 0 2 2.4 0 0 0 0 1 1]  GId=[66 66 47.6]  TcIF=[1 1 0.25 0.3 0 0 1 1 0.3 0.36 0 0 0 0]  GHd=[66 66 233]  TcHF="[0.01 0.012 0 0 0 0  0.012 0.0144 0 0 0 0 1 1]"  LIM=[.075 .15 .15 .15]  Plot_On=off  MagdB_On=off  FreqRange=logspace(-2,2,500)
      settings: LibrarySourceBlock=|
      | sps_lib/Electrical Machines/Synchronous Machine Control/Multi-Band
      | Power System Stabilizer
  Multiport Switch1 : MultiPortSwitch  Inputs=4  SaturateOnIntegerOverflow=off
  PSS model3 : Constant  Value=0
  PSS model4 : Constant
  Real-Imag to Complex1 : RealImagToComplex
  STG8 : spsSteamTurbineandGovernorLib/Steam Turbine and Governor  gentype=Tandem-compound (single mass)  reg1="[ 1  0.05    0 ]"  reg2="[ 0.001  0.15 ]"  reg3="[ -0.1  0.1  0  4.496 ]"  N=Ns  turb1="[ 0  10   3.3   0.5   ]"  turb2="[   0   0.36    0.36   0.28   ]"  HA="[ 0.046  1.430  1.465   0.192 ]"  KA="[ 90.44  53.88  64.59   62.94  ]"  DA="[ 0.0115  0.3575  0.3663   0.0137  ]"  ini1=0.54  ini2=[0.779316,-31.4247]
      settings: LibrarySourceBlock=|
      | sps_lib/Electrical Machines/Synchronous Machine Control/Steam Turbine
      | and Governor
  Sum2 : Sum  InputSameDT=on  SaturateOnIntegerOverflow=on  OutDataTypeStr=Inherit: Same as first input
  Sum3 : Sum  Inputs=-+  InputSameDT=on  SaturateOnIntegerOverflow=on  OutDataTypeStr=Inherit: Same as first input
  Terminator3 : Terminator
  Terminator4 : Terminator
  Terminator5 : Terminator
  wref8 : Constant
  Pm8 : Outport  InitialOutput=0
  Vf8 : Outport  Port=2  InitialOutput=0
  tag scope: EFD8=global, Pa8=global, Pe8=global, Q8=global, Vt8=global, d_theta8=global, pss8=global, theta8=global, w8=global
  wires:
  Bus Selector/7 -> EXCITATION8/3, Real-Imag to Complex1/2  "<Stator voltage  vq (pu)>"
  wref8/1 -> STG8/1
  Pref8/1 -> STG8/2
  m8/1 -> Bus Selector/1
  Vref8/1 -> EXCITATION8/1
  EXCITATION8/1 -> Vf8/1, [EFD8]
  Real-Imag to Complex1/1 -> [Vt8]
  Bus Selector/5 -> [theta8]  "<Rotor mechanical angle  theta (deg)>"
  Bus Selector/6 -> EXCITATION8/2, Real-Imag to Complex1/1  "<Stator voltage  vd (pu)>"
  STG8/3 -> Terminator3/1
  STG8/4 -> Sum3/2, Pm8/1
  STG8/2 -> Terminator4/1
  STG8/1 -> Terminator5/1
  Bus Selector/1 -> [w8], STG8/3  "<Rotor speed  wm  (pu)>"
  Bus Selector/2 -> STG8/4, [d_theta8]  "<Rotor angle deviation  d_theta (rad)>"
  Bus Selector/3 -> Sum3/1, [Pe8]  "<Electrical power  Pe (pu)>"
  Bus Selector/4 -> Delta w PSS (Kundur) 8/1, MB-PSS8/1  "<Rotor speed deviation  dw (pu)>"
  Bus Selector/8 -> [Q8]  "<Output reactive power  Qeo (pu)>"
  Sum3/1 -> [Pa8], "Delta Pa PSS 8 "/1  "Pm-Pe"
  Sum2/1 -> Multiport Switch1/1
  PSS model4/1 -> Sum2/2
  "Delta Pa PSS 8 "/1 -> Multiport Switch1/5
  Delta w PSS (Kundur) 8/1 -> Multiport Switch1/4
  MB-PSS8/1 -> Multiport Switch1/3
  PSS model3/1 -> Multiport Switch1/2
  Multiport Switch1/1 -> [pss8], EXCITATION8/4
  PSS8/1 -> Sum2/1

== system IEEE_BUS_68_AGC/area-3/G9/M9: Turbine & Regulators  ==
  note: M9
  m9 : Inport
  Pref9 : Inport  Port=2
  Vref9 : Inport  Port=3
  PSS9 : Inport  Port=4
  Bus Selector : BusSelector  OutputSignals="Mechanical.Rotor speed  wm  (pu),Mechanical.Rotor angle deviation  d_theta (rad),Mechanical.Electrical power  Pe (pu),Mechanical.Rotor speed deviation  dw (pu),Mechanical.Rotor mechanical angle  theta (deg),dq0 components.Stator voltage  vd (pu),dq0 components.Stator voltage  vq (pu),Output reactive power  Qeo (pu)"
  "Delta Pa PSS 9 " : spsGenericPowerSystemStabilizerLib/Generic Power System Stabilizer  Tsensor=15e-3  K=2.5*1.25  Twashout=1  Tleadlag1=[60e-3 1]  Tleadlag2=[0 0]  VSlimits=[-0.15 0.15]  Vinit=0  Plot_On=off  MagdB_On=on  FreqRange=logspace(-2,2,500)
      settings: LibrarySourceBlock=|
      | sps_lib/Electrical Machines/Synchronous Machine Control/Generic
      | Power System Stabilizer
  Delta w PSS (Kundur) 9 : spsGenericPowerSystemStabilizerLib/Generic Power System Stabilizer  Tsensor=15e-3  K=30  Twashout=10  Tleadlag1=[50e-3 20e-3]  Tleadlag2=[3 5.4]  VSlimits=[-0.15 0.15]  Vinit=0  Plot_On=off  MagdB_On=on  FreqRange=logspace(-2,2,500)
      settings: LibrarySourceBlock=|
      | sps_lib/Electrical Machines/Synchronous Machine Control/Generic
      | Power System Stabilizer
  EXCITATION9 : spsExcitationSystemLib/Excitation System  tr=AVR_Data(9,1)  reg=[ AVR_Data(9,2:3) ]  exc=[ 1, 0 ]  tgr=[ AVR_Data(9,4:5)]  damp=[ 0, 0 ]  sat=[ 0, 0 ]  lim="[ AVR_Data(9,7:8)  0 ]"  v0=[1.025 1.0445]
      settings: LibrarySourceBlock=sps_lib/Electrical Machines/Synchronous Machine Control/Excitation System
  MB-PSS9 : spsMultiBandPowerSystemStabilizerLib/Multi-Band Power System Stabilizer  OperationMode=Simplified settings  Kg=MB(1)  GL=[MB(2) MB(3)]  GI=[MB(4) MB(5)]  GH=[MB(6) MB(7)]  GLd=[66 66 9.4]  TcLF=[1.667 2 0 0 0 0 2 2.4 0 0 0 0 1 1]  GId=[66 66 47.6]  TcIF=[1 1 0.25 0.3 0 0 1 1 0.3 0.36 0 0 0 0]  GHd=[66 66 233]  TcHF="[0.01 0.012 0 0 0 0  0.012 0.0144 0 0 0 0 1 1]"  LIM=[.075 .15 .15 .15]  Plot_On=off  MagdB_On=off  FreqRange=logspace(-2,2,500)
      settings: LibrarySourceBlock=|
      | sps_lib/Electrical Machines/Synchronous Machine Control/Multi-Band
      | Power System Stabilizer
  Multiport Switch1 : MultiPortSwitch  Inputs=4  SaturateOnIntegerOverflow=off
  PSS model3 : Constant  Value=0
  PSS model4 : Constant
  Real-Imag to Complex1 : RealImagToComplex
  STG9 : spsSteamTurbineandGovernorLib/Steam Turbine and Governor  gentype=Tandem-compound (single mass)  reg1="[ 1  0.05    0 ]"  reg2="[ 0.001  0.15 ]"  reg3="[ -0.1  0.1  0  4.496 ]"  N=Ns  turb1="[ 0  10   3.3   0.5   ]"  turb2="[   0   0.36    0.36   0.28   ]"  HA="[ 0.046  1.430  1.465   0.192 ]"  KA="[ 90.44  53.88  64.59   62.94  ]"  DA="[ 0.0115  0.3575  0.3663   0.0137  ]"  ini1=0.8  ini2=[0.779316,-31.4247]
      settings: LibrarySourceBlock=|
      | sps_lib/Electrical Machines/Synchronous Machine Control/Steam Turbine
      | and Governor
  Sum2 : Sum  InputSameDT=on  SaturateOnIntegerOverflow=on  OutDataTypeStr=Inherit: Same as first input
  Sum3 : Sum  Inputs=-+  InputSameDT=on  SaturateOnIntegerOverflow=on  OutDataTypeStr=Inherit: Same as first input
  Terminator3 : Terminator
  Terminator4 : Terminator
  Terminator5 : Terminator
  wref9 : Constant
  Pm9 : Outport  InitialOutput=0
  Vf9 : Outport  Port=2  InitialOutput=0
  tag scope: EFD9=global, Pa9=global, Pe9=global, Q9=global, Vt9=global, d_theta9=global, pss9=global, theta9=global, w9=global
  wires:
  PSS9/1 -> Sum2/1
  Multiport Switch1/1 -> EXCITATION9/4, [pss9]
  PSS model3/1 -> Multiport Switch1/2
  MB-PSS9/1 -> Multiport Switch1/3
  Delta w PSS (Kundur) 9/1 -> Multiport Switch1/4
  "Delta Pa PSS 9 "/1 -> Multiport Switch1/5
  PSS model4/1 -> Sum2/2
  Sum2/1 -> Multiport Switch1/1
  Sum3/1 -> "Delta Pa PSS 9 "/1, [Pa9]  "Pm-Pe"
  Bus Selector/8 -> [Q9]  "<Output reactive power  Qeo (pu)>"
  Bus Selector/4 -> MB-PSS9/1, Delta w PSS (Kundur) 9/1  "<Rotor speed deviation  dw (pu)>"
  Bus Selector/3 -> [Pe9], Sum3/1  "<Electrical power  Pe (pu)>"
  Bus Selector/2 -> [d_theta9], STG9/4  "<Rotor angle deviation  d_theta (rad)>"
  Bus Selector/1 -> STG9/3, [w9]  "<Rotor speed  wm  (pu)>"
  STG9/1 -> Terminator5/1
  STG9/2 -> Terminator4/1
  STG9/4 -> Pm9/1, Sum3/2
  STG9/3 -> Terminator3/1
  Bus Selector/6 -> Real-Imag to Complex1/1, EXCITATION9/2  "<Stator voltage  vd (pu)>"
  Bus Selector/5 -> [theta9]  "<Rotor mechanical angle  theta (deg)>"
  Real-Imag to Complex1/1 -> [Vt9]
  EXCITATION9/1 -> [EFD9], Vf9/1
  Vref9/1 -> EXCITATION9/1
  m9/1 -> Bus Selector/1
  Pref9/1 -> STG9/2
  wref9/1 -> STG9/1
  Bus Selector/7 -> Real-Imag to Complex1/2, EXCITATION9/3  "<Stator voltage  vq (pu)>"
